simulink model "bpsk"  (Simulink 7.1)
settings: Solver=FixedStepDiscrete  StartTime=0.0  StopTime=10.0  FixedStep=0.001  RelTol=1e-3
libraries: dsPICdrivers x8, commdigbbndpm3 x2, commchan3 x1
settings Model: Creator=Liza  ModifiedByFormat=Liza  LastModifiedBy=Liza
settings OptimizationCC: OptimizeModelRefInitCode=on  LifeSpan=1
settings HardwareCC: ProdBitPerInt=16  ProdEndianess=LittleEndian  ProdWordSize=16  ProdHWDeviceType=16-bit Generic
settings RTWCC: SystemTargetFile=dspic.tlc  TemplateMakefile=dspic_pic30_gcc.tmf  PostCodeGenCommand=dsPIC_Compile()  Description=Embedded Target for Microchip dsPIC (real-time)  ProcessScript=dspic_make_rtw_hook
settings CodeAppCC: IgnoreCustomStorageClasses=off
settings STFCustomTargetCC: ModelReferenceCompliant=off  IncludeMdlTerminateFcn=off  CombineOutputUpdateFcns=on  SuppressErrorStatus=on  ERTCustomFileBanners=on  SupportContinuousTime=off  SupportNonInlinedSFcns=off  SystemTargetFile=dspic.tlc
settings ERTTargetCC: ModelReferenceCompliant=off  CompOptLevelCompliant=off  IncludeMdlTerminateFcn=off  SuppressErrorStatus=on  ERTFirstTimeCompliant=off  ModelStepFunctionPrototypeControlCompliant=off  InlinedParameterPlacement=NonHierarchical  ERTSrcFileBannerTemplate=dsPIC_code_template.cgt  ERTHdrFileBannerTemplate=dsPIC_code_template.cgt  ERTDataSrcFileTemplate=dsPIC_code_template.cgt  ERTDataHdrFileTemplate=dsPIC_code_template.cgt  ERTCustomFileTemplate=dsPIC_main.tlc
settings CustomProperty: DataType=string  Value=D:\PROGRA~1\MATLAB\R2008a\bin\win32\gmake

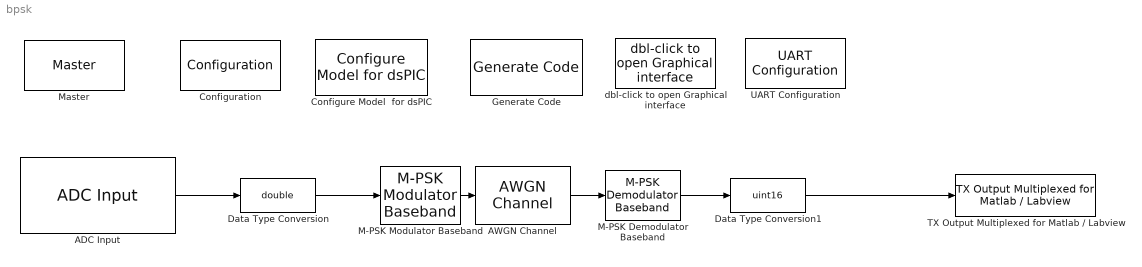
== system bpsk ==
  ADC Input : dsPICdrivers/Peripheral I//O/ADC Input  Tag=dsPIC_ADC  Priority=5  ADC_TYPE=12 bits  ADC_MODE=Continuous sampling & get last channel value  NbrSampleStep=1  VoltRefpopup="AVdd  -  AVss"  OutFormatBitspopup=0000 dddd dddd dddd : Integer  InterruptPriority=6  ANCHANNELS=[0 ]  MaxName=ANmax = 4095  Rin=1e2  ADCS=3  SAMC=1  Temperature=25  DMAChannel=0  SampleTime=.001  Status="OK  |  Tsmp=8.000e-007 |  T/Channel=1.200e-005 |  Tall=1.200e-005"  SSRC=auto convert
  AWGN Channel : commchan3/AWGN Channel  SystemSampleTime=-1  seed=67  noiseMode="Signal to noise ratio  (Eb/No)"  EbNodB=10  EsNodB=10  SNRdB=10  bitsPerSym=1  Ps=1  Tsym=1  variance=1
  Configuration : dsPICdrivers/Configuration  SystemSampleTime=-1  double64=off
  Configure Model  for dsPIC : dsPICdrivers/Simulink Configuration/Configure Model  for dsPIC
  Data Type Conversion : DataTypeConversion  OutDataTypeMode=double  OutDataType=sfix(16)  OutScaling=2^0  OutDataTypeStr=double
  Data Type Conversion1 : DataTypeConversion  OutDataTypeMode=uint16  OutDataType=sfix(16)  OutScaling=2^0  OutDataTypeStr=uint16
  Generate Code : dsPICdrivers/Simulink Configuration/Generate Code
  M-PSK Demodulator Baseband : commdigbbndpm3/M-PSK Demodulator Baseband  DialogController=commDDGCreate  DialogControllerArgs=DataTag0  M=2  Ph=pi  Dec=Binary  Mapping=[0:7]  OutType=Integer  DecType=Hard decision  VarSource=Dialog  Variance=1  outDtype1=Inherit via internal rule  outDtype2=Inherit via internal rule  derotateFactorWordLen=16
  M-PSK Modulator Baseband : commdigbbndpm3/M-PSK Modulator Baseband  M=2  InType=Integer  Enc=Binary  Mapping=0  Ph=0  outDtype=double  outWordLen=outWordLen  outUDDataType=outUDDataType  outFracLenMode=Best precision  outFracLen=outFracLen
  Master : dsPICdrivers/Master  Tag=dsPIC_MASTER  Priority=1  TimeStepType=Timer1  picType=30f2012  fcy=2.5e6  Quartz_33f=5e6  PLLActive_33f=off  fcyDesired_33f=0  tmr1="[1  4999  0]"  tmr1Info="Time Step : 0.001  ;   Error : 0%  PR1=2499"  tmr2345="[0  0]"  tmr2345cfg=[-1 -1]  IOautoConf=on  typePort="[ 0  0  0  0  0  0  0  0  0  0  0  0  0  0  0  0  8  0  0  0  0  0  0  0  0  0  0  0  0  0  0  0  0  0  0  0  0  0  0  0  0  0  0  0  0  5  4  0  0  0  0  0  0  0  0  0  0  0  0  0  0  0  0  0  0  0  0  0  0  0  0  0  0  0  0  0  0  0  0  0  0  0  0  0  0  0  0  0  0  0  0  0  0  0  0  0  0  0  0  0  0  0  0  0  0  0  0  0  0  0  0  0 ]"  TRIS="[ 65535  65535  65535  65535  65535  65535  65535 ]"  ADPCFG=0  MasterBusyPort=None  MasterOverloadPort=None  FOSC=HS  ClockSwitchMonitor=Both disabled  TempProtection_33f=TEMP_ON  FPBOR=PBOR_OFF  PWRT=PWRT_OFF  MCLR=MCLR_DIS  PowerSave=off  OverrideFcy=off  NewFcy=1e6  PR2345="[65535  65535]"
  TX Output Multiplexed for Matlab / Labview : dsPICdrivers/Serial PORT/TX Output Multiplexed for Matlab // Labview  Tag=dsPIC_TX_Multiplexed  Priority=5  UART=1  CleverSpreadingChk=on  CleverSpreading=1  CHANNEL=[0]  CHANNELBLOCKED=[]  CHANNELBLOCKED_BITEWISE=0  Status=OK
  UART Configuration : dsPICdrivers/Serial PORT/UART Configuration  Tag=dsPIC_config_UART  Priority=2  UART=1  proposed_BAUD=38400  ALT_TX_RX=on  InterruptTxWhen=When Transmit Buffer is empty  TXInterruptPri=1  TxBufferSize=32  TXEN=on  InterruptRxWhen=When Receive Buffer is full (contain 4 characters)  RXInterruptPri=2  RxBufferSize=32  BAUD=38400  UxBRG=3  Info="UxBRG = 3   ||  Real Baud : 39063   ||  % error : 1.7253  ||  max 3.9063 Bytes / Step"  RealBaud=0
  dbl-click to open Graphical interface : dsPICdrivers/Serial PORT/dbl-click to open Graphical interface  SystemSampleTime=-1  Nothing=0
  wires:
  ADC Input/1 -> Data Type Conversion/1
  Data Type Conversion1/1 -> TX Output Multiplexed for Matlab / Labview/1
  Data Type Conversion/1 -> M-PSK Modulator Baseband/1
  M-PSK Modulator Baseband/1 -> AWGN Channel/1
  AWGN Channel/1 -> M-PSK Demodulator Baseband/1
  M-PSK Demodulator Baseband/1 -> Data Type Conversion1/1
